simulink model "commhdlQPSKTxRxLoopback"  (R2025b)
settings: Solver=FixedStepDiscrete  StartTime=0.0  StopTime=0.03  RelTol=1e-3
PostLoadFcn:
  | hScopeConfig = get_param([gcs '/Receiver/QPSK Rx/Frequency and Time Synchronizer/Symbol Synchronizer/No HDL/QPSK Receiver Eye Diagram'],'ScopeConfiguration');
  | 
  | hScopeConfig.OpenAtSimulationStart = false;
  | hScopeConfig.Visible = false;
  | SamplesPerSymbol = 4;
  | %UpsamplesRx = 1;
  | clear hScopeConfig
InitFcn:
  | % RxAlign decoder latency (flat_simfix): 41 = netlist value used for HDL; set
  | % rxAlignLat = 25 in the base workspace before a model-level simulation.
  | if ~exist('rxAlignLat','var'), rxAlignLat = uint16(41); end
  | commhdlQPSKTxRxModelInit;
  | % Rate bridge: ADRV9002/Jupiter radio runs at 15.36 MHz = 2x the 7.68 MHz
  | % (4 samples/symbol @ Rsym=1.92 MHz) the QPSK Rx requires. The deployed
  | % Receiver must downsample the ADC stream by 2. UpsamplesRx=1 fed the QPSK
  | % Rx 8 sps (2x-upsampled) and broke symbol sync / the loopback bit check.
  | UpsamplesRx = 1;   %% T8 RATE FIX: rail 15.36e6 == ADC bus rate,
  | %% no ingress decimation (was 2 when the rail sat on the 7.68e6 rung)
  | UpsamplesTx = 1;
  | clear simTimingOffset;
StopFcn:
  | if exist('simTimingOffset','var')
  |   disp('Simulation completed');
  |   %QPSKTxRxVerification;
  | end
undefined symbols (not defined in the file or in its folder): Add, Config, fsym, randsrc, RandStream, Rsym, rxAlignLat, Shift
libraries: hdlsllib x141, simulink x45, dspsigops x30, dsphdlfiltering2 x6, dsphdlsigops2 x4, dsphdlmathfun2 x4, commdigbbndpm3 x4, dspmlti4 x2, commchan3 x1, commrflib2 x1, commcnvcod2 x1
(part 7 of 9)

== system commhdlQPSKTxRxLoopback/TxRxComposite/Receiver/QPSK Rx/Frequency and Time Synchronizer/Symbol Synchronizer/Rate Handle ==
  note: RATE HANDLE -- purpose
      | The Symbol Synchronizer's interpolator emits one symbol per timing-loop strobe, so its output is
      | valid on an IRREGULAR beat (the strobe drifts with the sample-rate offset and the timing correction).
      | Everything downstream (CFC, carrier sync, preamble detector, packet controller, demod) assumes a
      | REGULAR symbol stream: one valid in exactly 4 rail beats (sps = 4).  This block converts the former
      | to the latter with a small FIFO:
      |    push  = strobe            (dataIn is written whenever the interpolator produced a symbol)
      |    pop   = validIn & (phase == 0)   where phase is the free-running mod-4 HDL Counter
      | so validOut/dataOut are a 1-in-4 symbol stream and the FIFO absorbs the jitter between the two rates.
      | If the input runs slow the FIFO drains (EMPTY edge); if it runs fast it fills (FULL edge).  Those two
      | edges are the receiver's only rate-mismatch failure points, which is why every fix and instrument
      | in this subsystem watches or steers the pop.
      | Stock blocks: dataIn, strobe, validIn, Constant, FIFO, HDL Counter, Compare To Constant,
      | Logical Operator, dataOut, validOut.  Everything else was added by the overlay stack (notes below).
  note: bfGridEn / BfGridPace  (beatfix_overlay.m, fixctl 0x208 bit 2)
      | Selects which mod-4 phase counter drives the pop grid.  en = 0: the stock HDL Counter
      | (counts validIn beats).  en = 1: an absolute pacer that counts EVERY rail beat, so the pop
      | grid cannot slip when validIn drops out.  Default off = legacy-identical.
  note: Witness taps (read-only, no effect on the data path)
      | beatobsRhCtr / beatobsPush / beatobsPop  (beatobs_overlay.m): the mod-4 phase pointer and the FIFO
      |    push/pop pointers, routed up to the debug capture bus.
      | w1Strobe / w1Occ / w1PopEmpty / w1PushFull / w1PushPtr / w1PopPtr  (rxfix_w1_overlay.m): the W1 census
      |    inputs.  w1Occ is the FIFO's registered TRUE occupancy (not a pointer delta), counted by RxW1Census
      |    in the Frequency and Time Synchronizer into AXI 0x214-0x230 (0x220 = this block's validOut count).
  note: RxSteer -- pop steering  (rxfix_steer_overlay.m; formerly netlist variants R4B / R4D)
      | Keeps the FIFO away from its EMPTY and FULL edges by editing the pop, once per 13-slot window:
      |    window opens on sroPcEnd (Packet Controller endOut), lock after 8 windows
      |    occ <= 8   -> arm skipEn  : suppress one nominal pop        (EMPTY-edge guard, always on)
      |    occ >= 24  -> arm extraEn : insert one extra pop at phase 2 (FULL-edge guard, only if sroSign = 1)
      |    pop = (popNom & ~skipEn) | (extraEn & validIn & phase2 & sroSign)
      | sroSign is fixctl bit 5: 0 = R4B behaviour (148, negative SRO), 1 = R4D (146, positive SRO).
      | The pop expression is built from the AND/NOT/OR primitives OUTSIDE the MATLAB Function block, and
      | sroPcEnd / occ enter through Delay blocks, so HDL Coder cannot add a delay-match register that
      | would move the pop by a beat.  Witnesses: r4_wit 0x234 {locked, skips, opens}, r4_extras 0x238,
      | sro_mode 0x25C {extraArmed, sroSign}.
  dataIn : Inport
  strobe : Inport  Port=2
  validIn : Inport  Port=3
  bfGridEn : Inport  Port=4  OutDataTypeStr=boolean
  sroPcEnd : Inport  Port=5  OutDataTypeStr=boolean
  sroSign : Inport  Port=6  OutDataTypeStr=boolean
  BfGridPace : MATLAB Function  TreatAsAtomicUnit=on
  Compare To Constant : simulink/Logic and Bit Operations/Compare To Constant  relop===  const=0  OutDataTypeStr=boolean
  Constant : Constant  Value=false  SampleTime=-1
  FIFO : Subsystem  mask{fifoSize=32, pushFullDiag=Error, popEmptyDiag=Ignore}
      mask prompts: fifoSize "FIFO size:"; pushFullDiag "Push full FIFO:"; popEmptyDiag "Pop empty FIFO:"
      mask TypeOptions pushFullDiag: Ignore | Warning | Error
      mask TypeOptions popEmptyDiag: Ignore | Warning | Error
  HDL Counter : hdlsllib/Sources/HDL Counter  CountType=Count limited  CountInit=0  CountStep=1  CountMax=SamplesPerSymbol - 1  CountFromType=Initial value  CountFrom=0  CountResetPort=off  CountLoadPort=off  CountEnbPort=on  CountDirPort=off  CountHitOutputPort=off  CountDataType=Unsigned  CountWordLen=max(1, nextpow2(SamplesPerSymbol - 1))  CountFracLen=0  CountSampTime=1
  Logical Operator : Logic  AllPortsSameDT=off  OutDataTypeStr=boolean
  RxSteer : MATLAB Function  TreatAsAtomicUnit=on
  RxSteerDtcOcc : DataTypeConversion  OutDataTypeStr=uint8  ConvertRealWorld=Stored Integer (SI)  SaturateOnIntegerOverflow=off  RndMeth=Floor
  RxSteerExtraAnd : Logic  Inputs=4  AllPortsSameDT=off  OutDataTypeStr=boolean
  RxSteerNotSkip : Logic  Operator=NOT  Inputs=1  AllPortsSameDT=off  OutDataTypeStr=boolean
  RxSteerOccDly : Delay  DelayLength=1
  RxSteerOccFloor : simulink/Logic and Bit Operations/Compare To Constant  relop=>=  const=2  OutDataTypeStr=boolean
  RxSteerPhase2 : simulink/Logic and Bit Operations/Compare To Constant  relop===  const=1  OutDataTypeStr=boolean
  RxSteerPopOr : Logic  Operator=OR  AllPortsSameDT=off  OutDataTypeStr=boolean
  RxSteerSkipAnd : Logic  Inputs=3  AllPortsSameDT=off  OutDataTypeStr=boolean
  Terminator : Terminator
  dataOut : Outport
  validOut : Outport  Port=2
  beatobsRhCtr : Outport  Port=3
  beatobsPush : Outport  Port=4
  beatobsPop : Outport  Port=5
  w1Strobe : Outport  Port=6
  w1Occ : Outport  Port=7
  w1PopEmpty : Outport  Port=8
  w1PushFull : Outport  Port=9
  w1PushPtr : Outport  Port=10
  w1PopPtr : Outport  Port=11
  r4_wit : Outport  Port=12
  r4_extras : Outport  Port=13
  sro_mode : Outport  Port=14
  wires:
  RxSteerExtraAnd/1 -> RxSteerPopOr/2
  RxSteerNotSkip/1 -> RxSteerSkipAnd/2
  RxSteerOccFloor/1 -> RxSteerSkipAnd/3
  RxSteer/5(sroMode) -> sro_mode/1
  RxSteer/4(r4Extras) -> r4_extras/1
  RxSteerPhase2/1 -> RxSteer/4(phase2), RxSteerExtraAnd/3
  RxSteer/2(extraEn) -> RxSteerExtraAnd/1
  dataIn/1 -> FIFO/1(in)
  RxSteerSkipAnd/1 -> RxSteerPopOr/1
  RxSteerOccDly/1 -> RxSteerDtcOcc/1
  Logical Operator/1 -> RxSteerSkipAnd/1, RxSteer/2(popNom)
  validIn/1 -> HDL Counter/1, RxSteerExtraAnd/2, RxSteer/1(validIn), Logical Operator/1
  BfGridPace/1(y) -> beatobsRhCtr/1, Compare To Constant/1, RxSteerPhase2/1
  FIFO/3(validPop) -> validOut/1
  bfGridEn/1 -> BfGridPace/2(en)
  FIFO/2(numEntries) -> Terminator/1
  FIFO/1(out) -> dataOut/1
  RxSteerPopOr/1 -> FIFO/3(pop)
  Constant/1 -> FIFO/4(reset)
  FIFO/6(w1Occ) -> RxSteerOccDly/1, w1Occ/1
  RxSteer/3(r4Wit) -> r4_wit/1
  HDL Counter/1 -> BfGridPace/1(c)
  FIFO/4(beatobsPush) -> beatobsPush/1
  strobe/1 -> w1Strobe/1, FIFO/2(push)
  FIFO/7(w1PopEmpty) -> w1PopEmpty/1
  FIFO/5(beatobsPop) -> beatobsPop/1
  FIFO/8(w1PushFull) -> w1PushFull/1
  FIFO/9(w1PushPtr) -> w1PushPtr/1
  FIFO/10(w1PopPtr) -> w1PopPtr/1
  sroPcEnd/1 -> RxSteer/5(pcEnd)
  sroSign/1 -> RxSteer/6(sroSign), RxSteerExtraAnd/4
  RxSteerDtcOcc/1 -> RxSteerOccFloor/1, RxSteer/3(occ)
  Compare To Constant/1 -> Logical Operator/2
  RxSteer/1(skipEn) -> RxSteerNotSkip/1

== system commhdlQPSKTxRxLoopback/TxRxComposite/Transmitter/QPSK Tx/Bit Packetizer/Data Bits FIFO/No HDL ==
  push : Inport
  pop : Inport  Port=2
  MATLAB Function : MATLAB Function  TreatAsAtomicUnit=on
  No HDL : Subsystem
  wires:
  MATLAB Function/3(empty) -> No HDL/4(empty)
  MATLAB Function/2(ncount) -> No HDL/3(ncount)
  MATLAB Function/1(full) -> No HDL/2(full)
  pop/1 -> MATLAB Function/2(rd), No HDL/5(pop)
  push/1 -> MATLAB Function/1(wr), No HDL/1(push)

== system commhdlQPSKTxRxLoopback/TxRxComposite/Transmitter/QPSK Tx/Bit Packetizer/Preamble Bits Generator/Preamble Bits Store ==
  note: The Preamble is padded with zeros in the LUT such that
      | the length is the 2^nextpow2(length(Preamble)) for
      | efficient resource mapping to RAM
  actualPreamble : Inport
  sampleCount : Inport  Port=2
  Constant : Constant  OutDataTypeStr=boolean  SampleTime=1/(Rsym*SamplesPerSymbol)
  Extract Bits : simulink/Logic and Bit Operations/Extract Bits  bitsToExtract=Range of bits  numBits=8  bitIdxRange=[0 nextpow2(length(Preamble))-1]  outScalingMode=Treat bit field as an integer
  Preamble : LookupNDDirect  NumberOfTableDimensions=1  Table=[Preamble;false(32-length(Preamble),1)]  DiagnosticForOutOfRangeInput=Error
  Switch : Switch  Criteria=u2 ~= 0  Threshold=1  SaturateOnIntegerOverflow=off  InputSameDT=off
  preamble : Outport
  wires:
  Switch/1 -> preamble/1
  Constant/1 -> Switch/3
  actualPreamble/1 -> Switch/2
  Preamble/1 -> Switch/1
  Extract Bits/1 -> Preamble/1
  sampleCount/1 -> Extract Bits/1

== system commhdlQPSKTxRxLoopback/Receiver/QPSK Rx/Frequency and Time Synchronizer/Coarse Frequency Compensator/Coarse Frequency Estimator/Integrator/Reset Generator ==
  validIn : Inport
  Compare To Constant : simulink/Logic and Bit Operations/Compare To Constant  relop===  const=integAvgLen  OutDataTypeStr=boolean
  Delay1 : Delay  DelayLength=1
  Delay5 : Delay  DelayLength=1
  HDL Counter : hdlsllib/Sources/HDL Counter  CountType=Count limited  CountInit=0  CountStep=1  CountMax=integAvgLen  CountFromType=Initial value  CountFrom=0  CountResetPort=off  CountLoadPort=off  CountEnbPort=on  CountDirPort=off  CountHitOutputPort=off  CountDataType=Unsigned  CountWordLen=nextpow2(integAvgLen + 1)  CountFracLen=0  CountSampTime=1
  Logical Operator : Logic  AllPortsSameDT=off  OutDataTypeStr=boolean
  reset : Outport
  wires:
  Delay1/1 -> Logical Operator/1
  Delay5/1 -> Compare To Constant/1
  Logical Operator/1 -> reset/1
  validIn/1 -> HDL Counter/1, Delay1/1
  Compare To Constant/1 -> Logical Operator/2
  HDL Counter/1 -> Delay5/1

== system commhdlQPSKTxRxLoopback/Receiver/QPSK Rx/Frequency and Time Synchronizer/Phase Ambiguity Estimation and Correction/Phase Ambiguity Corrector/Reciprocal/Function Impl ==
  switch : Inport
  LUTAddr : Inport  Port=2
  Delay{6..8,10,15..16} (6 alike) : Delay
  Delay9 : Delay  DelayLength=1
  LUT1 : LookupNDDirect  NumberOfTableDimensions=1  Table=LUT(:,1)  DiagnosticForOutOfRangeInput=Error
  LUT2 : LookupNDDirect  NumberOfTableDimensions=1  Table=LUT(:,2)  DiagnosticForOutOfRangeInput=Error
  Multiport Switch : MultiPortSwitch  DataPortOrder=Zero-based contiguous  Inputs=2  zeroidx=on  SaturateOnIntegerOverflow=off  InputSameDT=off
  functionValues : Outport
  wires:
  Multiport Switch/1 -> Delay9/1
  Delay6/1 -> LUT1/1
  Delay7/1 -> LUT2/1
  Delay8/1 -> Delay10/1
  switch/1 -> Delay8/1
  LUT1/1 -> Delay16/1
  LUT2/1 -> Delay15/1
  Delay9/1 -> functionValues/1
  Delay10/1 -> Multiport Switch/1
  Delay16/1 -> Multiport Switch/3
  Delay15/1 -> Multiport Switch/2
  LUTAddr/1 -> Delay6/1, Delay7/1

== system commhdlQPSKTxRxLoopback/Receiver/QPSK Rx/Frequency and Time Synchronizer/Preamble Detector/FIFO/Validate Input Push Pop/No HDL ==
  pushFullFIFO : Inport
  popEmptyFIFO : Inport  Port=2
  Constant2 : Constant  Value=pushFullDiag  SampleTime=-1
  Constant3 : Constant  Value=popEmptyDiag  SampleTime=-1
  MATLAB Function : MATLAB Function  TreatAsAtomicUnit=on
  wires:
  Constant2/1 -> MATLAB Function/1(pushFullDiag)
  Constant3/1 -> MATLAB Function/2(popEmptyDiag)
  popEmptyFIFO/1 -> MATLAB Function/4(popEmpty)
  pushFullFIFO/1 -> MATLAB Function/3(pushFull)

== system commhdlQPSKTxRxLoopback/Receiver/QPSK Rx/Frequency and Time Synchronizer/Preamble Detector/Timing Adjust/No HDL/No HDL ==
  timingOffset : Inport
  Enable : EnablePort
  Data Type Conversion : DataTypeConversion  OutDataTypeStr=double  SaturateOnIntegerOverflow=off  RndMeth=Floor
  To Workspace : ToWorkspace  VariableName=simTimingOffset  SampleTime=-1
      settings: Save2DSignal=2-D array (concatenate along first dimension)
  wires:
  Data Type Conversion/1 -> To Workspace/1
  timingOffset/1 -> Data Type Conversion/1

== system commhdlQPSKTxRxLoopback/Receiver/QPSK Rx/Frequency and Time Synchronizer/Preamble Detector/Timing Adjust/No HDL/No HDL1 ==
  frameNumber : Inport
  Enable : EnablePort
  Data Type Conversion : DataTypeConversion  OutDataTypeStr=double  SaturateOnIntegerOverflow=off  RndMeth=Floor
  To Workspace : ToWorkspace  VariableName=simSyncedPackets  SampleTime=-1
      settings: Save2DSignal=2-D array (concatenate along first dimension)
  wires:
  frameNumber/1 -> Data Type Conversion/1
  Data Type Conversion/1 -> To Workspace/1

== system commhdlQPSKTxRxLoopback/Receiver/QPSK Rx/Frequency and Time Synchronizer/Symbol Synchronizer/Rate Handle/FIFO/Validate Input Push Pop ==
  rst : Inport
  push : Inport  Port=2
  pop : Inport  Port=3
  Compare To Constant : hdlsllib/Logic and Bit Operations/Compare To Constant  relop===  const=0  OutDataTypeStr=boolean
  Compare To Constant1 : hdlsllib/Logic and Bit Operations/Compare To Constant  relop===  const=fifoSize  OutDataTypeStr=boolean
  Constant : Constant  Value=true  SampleTime=-1
  Constant1 : Constant  Value=false  SampleTime=-1
  Delay : Delay  DelayLength=1
  Logical Operator1 : Logic  Operator=XOR  AllPortsSameDT=off  OutDataTypeStr=boolean
  Logical Operator2 : Logic  Operator=NOT  AllPortsSameDT=off  OutDataTypeStr=boolean
  Logical Operator{3..5,7,9} (5 alike) : Logic  AllPortsSameDT=off  OutDataTypeStr=boolean
  Logical Operator6 : Logic  Operator=NOT  AllPortsSameDT=off  OutDataTypeStr=boolean
  Logical Operator8 : Logic  Operator=NOT  AllPortsSameDT=off  OutDataTypeStr=boolean
  MATLAB Function : MATLAB Function  TreatAsAtomicUnit=on  mask{initVal=0, countToVal=fifoSize}
      mask prompts: initVal "Initial value:"; countToVal "Count to value:"
  No HDL : Subsystem
  Switch : Switch  Criteria=u2 ~= 0  SaturateOnIntegerOverflow=off  InputSameDT=off
  valid push : Outport
  valid pop : Outport  Port=2
  numEntries : Outport  Port=3
  wires:
  Logical Operator9/1 -> Logical Operator1/1, valid push/1
  Logical Operator2/1 -> Logical Operator9/2
  Logical Operator5/1 -> Logical Operator4/1
  Logical Operator8/1 -> Logical Operator5/2
  push/1 -> Logical Operator5/1, Logical Operator9/1
  Logical Operator1/1 -> MATLAB Function/2(enb)
  Logical Operator6/1 -> Logical Operator7/2
  Logical Operator7/1 -> Switch/2, valid pop/1, Logical Operator8/1, Logical Operator1/2
  Compare To Constant1/1 -> Logical Operator4/2
  Constant/1 -> Switch/3
  Logical Operator4/1 -> No HDL/1(pushFullFIFO), Logical Operator2/1  "push on full FIFO"
  Logical Operator3/1 -> No HDL/2(popEmptyFIFO), Logical Operator6/1  "pop on empty FIFO"
  Constant1/1 -> Switch/1
  MATLAB Function/1(count) -> Delay/1
  Switch/1 -> MATLAB Function/3(dir)
  pop/1 -> Logical Operator3/2, Logical Operator7/1
  Compare To Constant/1 -> Logical Operator3/1
  rst/1 -> MATLAB Function/1(rst)
  Delay/1 -> Compare To Constant1/1, numEntries/1, Compare To Constant/1

== system commhdlQPSKTxRxLoopback/TxRxComposite/Receiver/QPSK Rx/Frequency and Time Synchronizer/Coarse Frequency Compensator/Coarse Frequency Estimator/Extract Frequency ==
  datain : Inport
  validIn : Inport  Port=2
  Complex to Magnitude-Angle HDL Optimized : dsphdlmathfun2/Complex to Magnitude-Angle  NumIterationsSource=Auto  NumIterations=10  OutputFormat=Angle  AngleFormat=Normalized  ScaleOutput=on  ScalingMethod=Shift-Add  SimulateUsing=Code generation
  Delay{1..4} (4 alike) : Delay  DelayLength=1
  Gain : Gain  Gain=1/2  ParamDataTypeStr=fixdt(0,1,1)  OutDataTypeStr=Inherit: Same as input
  Unit Delay Enabled Synchronous : hdlsllib/Discrete/Unit Delay Enabled Synchronous  InitialCondition=0.0  SampleTime=-1
  normFreqOut : Outport
  wires:
  Delay3/1 -> normFreqOut/1
  Gain/1 -> Delay3/1
  Delay2/1 -> Gain/1
  Unit Delay Enabled Synchronous/1 -> Delay2/1
  Complex to Magnitude-Angle HDL Optimized/2 -> Unit Delay Enabled Synchronous/2
  Complex to Magnitude-Angle HDL Optimized/1 -> Unit Delay Enabled Synchronous/1
  Delay4/1 -> Complex to Magnitude-Angle HDL Optimized/2
  validIn/1 -> Delay4/1
  Delay1/1 -> Complex to Magnitude-Angle HDL Optimized/1
  datain/1 -> Delay1/1

== system commhdlQPSKTxRxLoopback/TxRxComposite/Receiver/QPSK Rx/Frequency and Time Synchronizer/Coarse Frequency Compensator/Coarse Frequency Estimator/Integrator ==
  note: store the value in the Reg before reset
  dataIn : Inport
  validIn : Inport  Port=2
  Add1 : Sum  Inputs=|++  OutDataTypeStr=Inherit: Same as first input
  Delay : Delay  DelayLength=1
  Delay1 : Delay  DelayLength=1
  Delay2 : Delay  DelayLength=1
  Integ Reg : hdlsllib/Discrete/Unit Delay Enabled Resettable Synchronous  InitialCondition=0.0  SampleTime=-1
  Reset Generator : Subsystem
  Store Reg : hdlsllib/Discrete/Unit Delay Enabled Synchronous  InitialCondition=0.0  SampleTime=-1
  IntegOut : Outport
  IntegValid : Outport  Port=2
  wires:
  Add1/1 -> Integ Reg/1
  Store Reg/1 -> IntegOut/1
  Delay1/1 -> Add1/1
  Delay/1 -> IntegValid/1
  Integ Reg/1 -> Store Reg/1, Add1/2
  Delay2/1 -> Integ Reg/2
  dataIn/1 -> Delay1/1
  Reset Generator/1(reset) -> Integ Reg/3, Delay/1, Store Reg/2
  validIn/1 -> Delay2/1, Reset Generator/1(validIn)

== system commhdlQPSKTxRxLoopback/TxRxComposite/Receiver/QPSK Rx/Frequency and Time Synchronizer/Phase Ambiguity Estimation and Correction/Phase Ambiguity Corrector/Reciprocal ==
  dataIn : Inport
  Compare To Constant : simulink/Logic and Bit Operations/Compare To Constant  relop=<  const=0  OutDataTypeStr=boolean
  Data Type Conversion : DataTypeConversion  OutDataTypeStr=fixdt(1,WL,0)  ConvertRealWorld=Stored Integer (SI)  SaturateOnIntegerOverflow=off  RndMeth=Floor
  Data Type Conversion1 : DataTypeConversion  OutDataTypeStr=fixdt(0,LUTAddrWL,0)  ConvertRealWorld=Stored Integer (SI)  SaturateOnIntegerOverflow=off  RndMeth=Floor
  Data Type Conversion2 : DataTypeConversion  OutDataTypeStr=fixdt(0,WL-LUTAddrWL,0)  ConvertRealWorld=Stored Integer (SI)  SaturateOnIntegerOverflow=off  RndMeth=Floor
  Delay : Delay  DelayLength=1
  Delay1 : Delay  DelayLength=1
  Delay2 : Delay  DelayLength=1
  Extract Bits : simulink/Logic and Bit Operations/Extract Bits  bitsToExtract=Range ending with least significant bit  numBits=LUTAddrWL  bitIdxRange=[0 7]  outScalingMode=Treat bit field as an integer
  Function Impl : Subsystem
  dataOut : Outport
  wires:
  Data Type Conversion1/1 -> Function Impl/2(LUTAddr)
  Data Type Conversion2/1 -> Function Impl/1(switch)
  Delay2/1 -> Data Type Conversion1/1
  Delay1/1 -> Data Type Conversion2/1
  Function Impl/1(functionValues) -> dataOut/1
  Delay/1 -> Compare To Constant/1, Extract Bits/1
  Compare To Constant/1 -> Delay1/1
  Data Type Conversion/1 -> Delay/1
  Extract Bits/1 -> Delay2/1
  dataIn/1 -> Data Type Conversion/1

== system commhdlQPSKTxRxLoopback/TxRxComposite/Receiver/QPSK Rx/Frequency and Time Synchronizer/Phase Ambiguity Estimation and Correction/Phase Ambiguity Estimator/Subsystem ==
  L : Inport
  H : Inport  Port=2
  Delay6 : Delay  DelayLength=1  InitialCondition=1
  Logical Operator : Logic  AllPortsSameDT=off  OutDataTypeStr=boolean
  Logical Operator1 : Logic  Operator=NOT  IconShape=distinctive  AllPortsSameDT=off  OutDataTypeStr=boolean
  Logical Operator2 : Logic  Operator=OR  AllPortsSameDT=off  OutDataTypeStr=boolean
  Out2 : Outport
  wires:
  Logical Operator/1 -> Logical Operator2/2
  Delay6/1 -> Out2/1, Logical Operator/2
  Logical Operator1/1 -> Logical Operator/1
  Logical Operator2/1 -> Delay6/1
  L/1 -> Logical Operator1/1
  H/1 -> Logical Operator2/1

== system commhdlQPSKTxRxLoopback/TxRxComposite/Receiver/QPSK Rx/Frequency and Time Synchronizer/Phase Ambiguity Estimation and Correction/Phase Ambiguity Estimator/Subsystem1 ==
  In1 : Inport
  validIn : Inport  Port=2
  Logical Operator1 : Logic  IconShape=distinctive  AllPortsSameDT=off  OutDataTypeStr=boolean
  Logical Operator2 : Logic  Operator=NOT  IconShape=distinctive  AllPortsSameDT=off  OutDataTypeStr=boolean
  validOut : Outport
  wires:
  validIn/1 -> Logical Operator1/2
  Logical Operator1/1 -> validOut/1
  Logical Operator2/1 -> Logical Operator1/1
  In1/1 -> Logical Operator2/1

== system commhdlQPSKTxRxLoopback/TxRxComposite/Receiver/QPSK Rx/Frequency and Time Synchronizer/Preamble Detector/Correlator/Magnitude Squared ==
  In1 : Inport
  Delay1 : Delay
  Delay2 : Delay
  Delay3 : Delay
  Math Function : Math  Operator=conj
  Product : Product
  Out1 : Outport
  wires:
  Delay3/1 -> Out1/1
  Product/1 -> Delay3/1
  Delay1/1 -> Product/2
  Delay2/1 -> Product/1
  Math Function/1 -> Delay1/1
  In1/1 -> Math Function/1, Delay2/1

== system commhdlQPSKTxRxLoopback/TxRxComposite/Receiver/QPSK Rx/Frequency and Time Synchronizer/Preamble Detector/Correlator/Magnitude Squared and Moving Sum ==
  scaled1 : Inport
  validIn : Inport  Port=2
  Add : Sum  Inputs=|+-  OutDataTypeStr=Inherit: Same as first input
  Add1 : Sum  Inputs=|++  OutDataTypeStr=Inherit: Same as first input
  Complex to Real-Imag1 : ComplexToRealImag  Output=Real
  Delay : Delay  DelayLength=26  ShowEnablePort=on
      settings: InputPortMap=u0,e6
  Delay{1..4,6,8..10,12} (9 alike) : Delay
  Delay11 : Delay  DelayLength=24
  Delay14 : Delay  DelayLength=1  ShowEnablePort=on
      settings: InputPortMap=u0,e6
  Delay5 : Delay  DelayLength=1
  Delay7 : Delay  DelayLength=1
  Gain : Gain  Gain=ThresoldGainFac  OutDataTypeStr=Inherit: Same as input
  Math Function1 : Math  Operator=conj
  Product1 : Product
  E1 : Outport
  wires:
  Delay11/1 -> E1/1
  Delay5/1 -> Add1/1
  Add/1 -> Delay5/1
  Delay/1 -> Add/2
  Delay4/1 -> Delay/1, Add/1
  Delay8/1 -> Delay/2, Delay7/1
  scaled1/1 -> Math Function1/1, Delay6/1
  Gain/1 -> Delay4/1
  validIn/1 -> Delay12/1
  Delay6/1 -> Product1/1
  Delay7/1 -> Delay14/2
  Math Function1/1 -> Delay1/1
  Product1/1 -> Delay2/1
  Delay10/1 -> Delay9/1
  Delay3/1 -> Gain/1
  Add1/1 -> Delay11/1, Delay14/1
  Delay1/1 -> Product1/2
  Delay14/1 -> Add1/2
  Delay9/1 -> Delay8/1
  Delay2/1 -> Complex to Real-Imag1/1
  Complex to Real-Imag1/1 -> Delay3/1
  Delay12/1 -> Delay10/1

== system commhdlQPSKTxRxLoopback/TxRxComposite/Receiver/QPSK Rx/Frequency and Time Synchronizer/Preamble Detector/FIFO/Validate Input Push Pop ==
  rst : Inport
  push : Inport  Port=2
  pop : Inport  Port=3
  Compare To Constant : hdlsllib/Logic and Bit Operations/Compare To Constant  relop===  const=0  OutDataTypeStr=boolean
  Compare To Constant1 : hdlsllib/Logic and Bit Operations/Compare To Constant  relop===  const=fifoSize  OutDataTypeStr=boolean
  Constant : Constant  Value=true  SampleTime=-1
  Constant1 : Constant  Value=false  SampleTime=-1
  Delay : Delay  DelayLength=1
  Logical Operator1 : Logic  Operator=XOR  AllPortsSameDT=off  OutDataTypeStr=boolean
  Logical Operator2 : Logic  Operator=NOT  AllPortsSameDT=off  OutDataTypeStr=boolean
  Logical Operator{3..5,7,9} (5 alike) : Logic  AllPortsSameDT=off  OutDataTypeStr=boolean
  Logical Operator6 : Logic  Operator=NOT  AllPortsSameDT=off  OutDataTypeStr=boolean
  Logical Operator8 : Logic  Operator=NOT  AllPortsSameDT=off  OutDataTypeStr=boolean
  MATLAB Function : MATLAB Function  TreatAsAtomicUnit=on  mask{initVal=0, countToVal=fifoSize}
      mask prompts: initVal "Initial value:"; countToVal "Count to value:"
  No HDL : Subsystem
  Switch : Switch  Criteria=u2 ~= 0  SaturateOnIntegerOverflow=off  InputSameDT=off
  valid push : Outport
  valid pop : Outport  Port=2
  numEntries : Outport  Port=3
  wires:
  Logical Operator3/1 -> No HDL/2(popEmptyFIFO), Logical Operator6/1  "pop on empty FIFO"
  Logical Operator4/1 -> No HDL/1(pushFullFIFO), Logical Operator2/1  "push on full FIFO"
  Compare To Constant/1 -> Logical Operator3/1
  Compare To Constant1/1 -> Logical Operator4/2
  Delay/1 -> Compare To Constant/1, Compare To Constant1/1, numEntries/1
  Logical Operator6/1 -> Logical Operator7/2
  push/1 -> Logical Operator9/1, Logical Operator5/1
  Logical Operator1/1 -> MATLAB Function/2(enb)
  Constant1/1 -> Switch/1
  pop/1 -> Logical Operator7/1, Logical Operator3/2
  rst/1 -> MATLAB Function/1(rst)
  Logical Operator8/1 -> Logical Operator5/2
  Switch/1 -> MATLAB Function/3(dir)
  Logical Operator2/1 -> Logical Operator9/2
  Logical Operator7/1 -> Switch/2, Logical Operator8/1, valid pop/1, Logical Operator1/2
  Logical Operator9/1 -> Logical Operator1/1, valid push/1
  MATLAB Function/1(count) -> Delay/1
  Constant/1 -> Switch/3
  Logical Operator5/1 -> Logical Operator4/1

== system commhdlQPSKTxRxLoopback/TxRxComposite/Receiver/QPSK Rx/Frequency and Time Synchronizer/Preamble Detector/Timing Adjust/No HDL ==
  note: This subsystem generates variables required for QPSKRxVerification for validation
  validIn : Inport
  timingOffset : Inport  Port=2
  syncPulse : Inport  Port=3
  Compare To Constant : simulink/Logic and Bit Operations/Compare To Constant  relop===  const=0  OutDataTypeStr=boolean
  Delay : Delay  DelayLength=4
  Delay1 : Delay  DelayLength=4
  Frame Counter : hdlsllib/Sources/HDL Counter  CountType=Free running  CountInit=0  CountStep=1  CountMax=bitsPerPacket/2 - 1  CountFromType=Initial value  CountFrom=0  CountResetPort=off  CountLoadPort=off  CountEnbPort=on  CountDirPort=off  CountHitOutputPort=off  CountDataType=Unsigned  CountWordLen=32  CountFracLen=0  CountSampTime=1
  Logical Operator : Logic  AllPortsSameDT=off  OutDataTypeStr=boolean
  No HDL : Subsystem
  No HDL1 : Subsystem
  Symbol Counter : hdlsllib/Sources/HDL Counter  CountType=Count limited  CountInit=0  CountStep=1  CountMax=bitsPerPacket/2 - 1  CountFromType=Initial value  CountFrom=0  CountResetPort=off  CountLoadPort=off  CountEnbPort=on  CountDirPort=off  CountHitOutputPort=off  CountDataType=Unsigned  CountWordLen=nextpow2(bitsPerPacket/2 - 1)  CountFracLen=0  CountSampTime=1
  Unit Delay Enabled Synchronous : hdlsllib/Discrete/Unit Delay Enabled Synchronous  InitialCondition=0.0  SampleTime=-1
  wires:
  Delay/1 -> No HDL1/Enable, No HDL/Enable
  Delay1/1 -> No HDL/1(timingOffset)
  timingOffset/1 -> Delay1/1
  Unit Delay Enabled Synchronous/1 -> No HDL1/1(frameNumber)
  Frame Counter/1 -> Unit Delay Enabled Synchronous/1
  Logical Operator/1 -> Frame Counter/1, Unit Delay Enabled Synchronous/2
  Symbol Counter/1 -> Compare To Constant/1
  syncPulse/1 -> Delay/1
  Compare To Constant/1 -> Logical Operator/1
  validIn/1 -> Symbol Counter/1, Logical Operator/2

== system commhdlQPSKTxRxLoopback/TxRxComposite/Receiver/QPSK Rx/Frequency and Time Synchronizer/Symbol Synchronizer/Gardner TED/GTED ==
  In1 : Inport
  Add : Sum
  Add1 : Sum  Inputs=+-
  Add2 : Sum  Inputs=+-
  Complex to Real-Imag : ComplexToRealImag
  Delay{,1,4..5,8,11} (6 alike) : Delay  DelayLength=1
  Delay{9..10,12..13} (4 alike) : Delay
  Product : Product
  Product1 : Product
  Out1 : Outport
  wires:
  Add/1 -> Out1/1
  Delay13/1 -> Add/2
  Delay10/1 -> Add/1
  Product/1 -> Delay10/1
  Complex to Real-Imag/2 -> Delay4/1, Add2/2
  Delay8/1 -> Product/1
  Add1/1 -> Delay9/1
  Delay/1 -> Delay1/1
  Product1/1 -> Delay13/1
  In1/1 -> Complex to Real-Imag/1
  Delay4/1 -> Delay5/1
  Delay1/1 -> Delay8/1, Add1/1
  Delay5/1 -> Add2/1, Delay11/1
  Add2/1 -> Delay12/1
  Delay9/1 -> Product/2
  Delay11/1 -> Product1/1
  Complex to Real-Imag/1 -> Delay/1, Add1/2
  Delay12/1 -> Product1/2

== system commhdlQPSKTxRxLoopback/TxRxComposite/Receiver/QPSK Rx/Frequency and Time Synchronizer/Symbol Synchronizer/No HDL/No HDL ==
  data : Inport
  Enable : EnablePort
  Data Type Conversion : DataTypeConversion  OutDataTypeStr=double  SaturateOnIntegerOverflow=off  RndMeth=Floor
  wires:
  Data Type Conversion/1 -> ?
  data/1 -> Data Type Conversion/1

== system commhdlQPSKTxRxLoopback/TxRxComposite/Receiver/QPSK Rx/Frequency and Time Synchronizer/Symbol Synchronizer/Rate Handle/FIFO ==
  in : Inport
  push : Inport  Port=2
  pop : Inport  Port=3
  reset : Inport  Port=4
  Delay1 : Delay  DelayLength=1
  Pop Counter : hdlsllib/Sources/HDL Counter  CountType=Count limited  CountInit=0  CountStep=1  CountMax=fifoSize -1  CountFromType=Initial value  CountFrom=0  CountResetPort=on  CountLoadPort=off  CountEnbPort=on  CountDirPort=off  CountHitOutputPort=off  CountDataType=Unsigned  CountWordLen=nextpow2(fifoSize)  CountFracLen=0  CountSampTime=1
  Push Counter : hdlsllib/Sources/HDL Counter  CountType=Count limited  CountInit=0  CountStep=1  CountMax=fifoSize -1  CountFromType=Initial value  CountFrom=0  CountResetPort=on  CountLoadPort=off  CountEnbPort=on  CountDirPort=off  CountHitOutputPort=off  CountDataType=Unsigned  CountWordLen=nextpow2(fifoSize)  CountFracLen=0  CountSampTime=1
  Simple Dual Port RAM : hdlsllib/HDL RAMs/Simple Dual Port RAM  ram_size=nextpow2(fifoSize)
  Validate Input Push Pop : Subsystem
  out : Outport
  numEntries : Outport  Port=2
  validPop : Outport  Port=3
  beatobsPush : Outport  Port=4
  beatobsPop : Outport  Port=5
  w1Occ : Outport  Port=6
  w1PopEmpty : Outport  Port=7
  w1PushFull : Outport  Port=8
  w1PushPtr : Outport  Port=9
  w1PopPtr : Outport  Port=10
  wires:
  Simple Dual Port RAM/1 -> out/1
  reset/1 -> Validate Input Push Pop/1(rst), Delay1/1
  Validate Input Push Pop/6(w1PushFull) -> w1PushFull/1
  push/1 -> Validate Input Push Pop/2(push)
  pop/1 -> Validate Input Push Pop/3(pop)
  Delay1/1 -> Push Counter/1, Pop Counter/1
  Validate Input Push Pop/3(numEntries) -> numEntries/1
  Validate Input Push Pop/1(valid push) -> Push Counter/2, Simple Dual Port RAM/3
  Validate Input Push Pop/4(w1Occ) -> w1Occ/1
  Validate Input Push Pop/5(w1PopEmpty) -> w1PopEmpty/1
  Validate Input Push Pop/2(valid pop) -> Pop Counter/2, validPop/1
  Push Counter/1 -> w1PushPtr/1, beatobsPush/1, Simple Dual Port RAM/2
  Pop Counter/1 -> w1PopPtr/1, beatobsPop/1, Simple Dual Port RAM/4
  in/1 -> Simple Dual Port RAM/1

== system commhdlQPSKTxRxLoopback/TxRxComposite/Transmitter/QPSK Tx/Bit Packetizer/Data Bits FIFO/No HDL/No HDL ==
  push : Inport
  full : Inport  Port=2
  ncount : Inport  Port=3
  empty : Inport  Port=4
  pop : Inport  Port=5
  Assertion : Assertion
  Assertion1 : Assertion
  Display : Display
  Logical Operator : Logic  Operator=NAND  AllPortsSameDT=off  OutDataTypeStr=boolean
  Logical Operator1 : Logic  Operator=NAND  AllPortsSameDT=off  OutDataTypeStr=boolean
  wires:
  Logical Operator1/1 -> Assertion1/1
  pop/1 -> Logical Operator1/2
  Logical Operator/1 -> Assertion/1
  empty/1 -> Logical Operator1/1
  full/1 -> Logical Operator/2
  push/1 -> Logical Operator/1
  ncount/1 -> Display/1

== system commhdlQPSKTxRxLoopback/Receiver/QPSK Rx/Frequency and Time Synchronizer/Symbol Synchronizer/Rate Handle/FIFO/Validate Input Push Pop/No HDL ==
  pushFullFIFO : Inport
  popEmptyFIFO : Inport  Port=2
  Constant2 : Constant  Value=pushFullDiag  SampleTime=-1
  Constant3 : Constant  Value=popEmptyDiag  SampleTime=-1
  MATLAB Function : MATLAB Function  TreatAsAtomicUnit=on
  wires:
  Constant2/1 -> MATLAB Function/1(pushFullDiag)
  Constant3/1 -> MATLAB Function/2(popEmptyDiag)
  popEmptyFIFO/1 -> MATLAB Function/4(popEmpty)
  pushFullFIFO/1 -> MATLAB Function/3(pushFull)

== system commhdlQPSKTxRxLoopback/TxRxComposite/Receiver/QPSK Rx/Frequency and Time Synchronizer/Coarse Frequency Compensator/Coarse Frequency Estimator/Integrator/Reset Generator ==
  validIn : Inport
  Compare To Constant : simulink/Logic and Bit Operations/Compare To Constant  relop===  const=integAvgLen  OutDataTypeStr=boolean
  Delay1 : Delay  DelayLength=1
  Delay5 : Delay  DelayLength=1
  HDL Counter : hdlsllib/Sources/HDL Counter  CountType=Count limited  CountInit=0  CountStep=1  CountMax=integAvgLen  CountFromType=Initial value  CountFrom=0  CountResetPort=off  CountLoadPort=off  CountEnbPort=on  CountDirPort=off  CountHitOutputPort=off  CountDataType=Unsigned  CountWordLen=nextpow2(integAvgLen + 1)  CountFracLen=0  CountSampTime=1
  Logical Operator : Logic  AllPortsSameDT=off  OutDataTypeStr=boolean
  reset : Outport
  wires:
  Logical Operator/1 -> reset/1
  Delay5/1 -> Compare To Constant/1
  Compare To Constant/1 -> Logical Operator/2
  Delay1/1 -> Logical Operator/1
  HDL Counter/1 -> Delay5/1
  validIn/1 -> HDL Counter/1, Delay1/1

== system commhdlQPSKTxRxLoopback/TxRxComposite/Receiver/QPSK Rx/Frequency and Time Synchronizer/Phase Ambiguity Estimation and Correction/Phase Ambiguity Corrector/Reciprocal/Function Impl ==
  switch : Inport
  LUTAddr : Inport  Port=2
  Delay{6..8,10,15..16} (6 alike) : Delay
  Delay9 : Delay  DelayLength=1
  LUT1 : LookupNDDirect  NumberOfTableDimensions=1  Table=LUT(:,1)  DiagnosticForOutOfRangeInput=Error
  LUT2 : LookupNDDirect  NumberOfTableDimensions=1  Table=LUT(:,2)  DiagnosticForOutOfRangeInput=Error
  Multiport Switch : MultiPortSwitch  DataPortOrder=Zero-based contiguous  Inputs=2  zeroidx=on  SaturateOnIntegerOverflow=off  InputSameDT=off
  functionValues : Outport
  wires:
  Delay9/1 -> functionValues/1
  Delay10/1 -> Multiport Switch/1
  LUT1/1 -> Delay16/1
  LUT2/1 -> Delay15/1
  Delay8/1 -> Delay10/1
  Multiport Switch/1 -> Delay9/1
  Delay6/1 -> LUT1/1
  Delay16/1 -> Multiport Switch/3
  Delay15/1 -> Multiport Switch/2
  Delay7/1 -> LUT2/1
  switch/1 -> Delay8/1
  LUTAddr/1 -> Delay6/1, Delay7/1

== system commhdlQPSKTxRxLoopback/TxRxComposite/Receiver/QPSK Rx/Frequency and Time Synchronizer/Preamble Detector/FIFO/Validate Input Push Pop/No HDL ==
  pushFullFIFO : Inport
  popEmptyFIFO : Inport  Port=2
  Constant2 : Constant  Value=pushFullDiag  SampleTime=-1
  Constant3 : Constant  Value=popEmptyDiag  SampleTime=-1
  MATLAB Function : MATLAB Function  TreatAsAtomicUnit=on
  wires:
  pushFullFIFO/1 -> MATLAB Function/3(pushFull)
  popEmptyFIFO/1 -> MATLAB Function/4(popEmpty)
  Constant3/1 -> MATLAB Function/2(popEmptyDiag)
  Constant2/1 -> MATLAB Function/1(pushFullDiag)

== system commhdlQPSKTxRxLoopback/TxRxComposite/Receiver/QPSK Rx/Frequency and Time Synchronizer/Preamble Detector/Timing Adjust/No HDL/No HDL ==
  timingOffset : Inport
  Enable : EnablePort
  Data Type Conversion : DataTypeConversion  OutDataTypeStr=double  SaturateOnIntegerOverflow=off  RndMeth=Floor
  wires:
  timingOffset/1 -> Data Type Conversion/1

== system commhdlQPSKTxRxLoopback/TxRxComposite/Receiver/QPSK Rx/Frequency and Time Synchronizer/Preamble Detector/Timing Adjust/No HDL/No HDL1 ==
  frameNumber : Inport
  Enable : EnablePort
  Data Type Conversion : DataTypeConversion  OutDataTypeStr=double  SaturateOnIntegerOverflow=off  RndMeth=Floor
  wires:
  frameNumber/1 -> Data Type Conversion/1

== system commhdlQPSKTxRxLoopback/TxRxComposite/Receiver/QPSK Rx/Frequency and Time Synchronizer/Symbol Synchronizer/Rate Handle/FIFO/Validate Input Push Pop ==
  rst : Inport
  push : Inport  Port=2
  pop : Inport  Port=3
  Compare To Constant : hdlsllib/Logic and Bit Operations/Compare To Constant  relop===  const=0  OutDataTypeStr=boolean
  Compare To Constant1 : hdlsllib/Logic and Bit Operations/Compare To Constant  relop===  const=fifoSize  OutDataTypeStr=boolean
  Constant : Constant  Value=true  SampleTime=-1
  Constant1 : Constant  Value=false  SampleTime=-1
  Delay : Delay  DelayLength=1
  Logical Operator1 : Logic  Operator=XOR  AllPortsSameDT=off  OutDataTypeStr=boolean
  Logical Operator2 : Logic  Operator=NOT  AllPortsSameDT=off  OutDataTypeStr=boolean
  Logical Operator{3..5,7,9} (5 alike) : Logic  AllPortsSameDT=off  OutDataTypeStr=boolean
  Logical Operator6 : Logic  Operator=NOT  AllPortsSameDT=off  OutDataTypeStr=boolean
  Logical Operator8 : Logic  Operator=NOT  AllPortsSameDT=off  OutDataTypeStr=boolean
  MATLAB Function : MATLAB Function  TreatAsAtomicUnit=on  mask{initVal=0, countToVal=fifoSize}
      mask prompts: initVal "Initial value:"; countToVal "Count to value:"
  No HDL : Subsystem
  Switch : Switch  Criteria=u2 ~= 0  SaturateOnIntegerOverflow=off  InputSameDT=off
  valid push : Outport
  valid pop : Outport  Port=2
  numEntries : Outport  Port=3
  w1Occ : Outport  Port=4
  w1PopEmpty : Outport  Port=5
  w1PushFull : Outport  Port=6
  wires:
  Compare To Constant/1 -> Logical Operator3/1
  Logical Operator4/1 -> w1PushFull/1, No HDL/1(pushFullFIFO), Logical Operator2/1  "push on full FIFO"
  Delay/1 -> w1Occ/1, Compare To Constant/1, Compare To Constant1/1, numEntries/1
  Logical Operator6/1 -> Logical Operator7/2
  Logical Operator3/1 -> w1PopEmpty/1, No HDL/2(popEmptyFIFO), Logical Operator6/1  "pop on empty FIFO"
  push/1 -> Logical Operator9/1, Logical Operator5/1
  Logical Operator5/1 -> Logical Operator4/1
  pop/1 -> Logical Operator7/1, Logical Operator3/2
  Logical Operator9/1 -> Logical Operator1/1, valid push/1
  Logical Operator7/1 -> Switch/2, valid pop/1, Logical Operator1/2, Logical Operator8/1
  Constant1/1 -> Switch/1
  Constant/1 -> Switch/3
  rst/1 -> MATLAB Function/1(rst)
  Compare To Constant1/1 -> Logical Operator4/2
  Logical Operator1/1 -> MATLAB Function/2(enb)
  Logical Operator2/1 -> Logical Operator9/2
  Switch/1 -> MATLAB Function/3(dir)
  Logical Operator8/1 -> Logical Operator5/2
  MATLAB Function/1(count) -> Delay/1

== system commhdlQPSKTxRxLoopback/TxRxComposite/Receiver/QPSK Rx/Frequency and Time Synchronizer/Symbol Synchronizer/Rate Handle/FIFO/Validate Input Push Pop/No HDL ==
  pushFullFIFO : Inport
  popEmptyFIFO : Inport  Port=2
  Constant2 : Constant  Value=pushFullDiag  SampleTime=-1
  Constant3 : Constant  Value=popEmptyDiag  SampleTime=-1
  MATLAB Function : MATLAB Function  TreatAsAtomicUnit=on
  wires:
  pushFullFIFO/1 -> MATLAB Function/3(pushFull)
  popEmptyFIFO/1 -> MATLAB Function/4(popEmpty)
  Constant3/1 -> MATLAB Function/2(popEmptyDiag)
  Constant2/1 -> MATLAB Function/1(pushFullDiag)

== matlab function commhdlQPSKTxRxLoopback/Receiver/QPSK Rx/Frequency and Time Synchronizer/Symbol Synchronizer/Rate Handle/FIFO/Validate Input Push Pop/No HDL/MATLAB Function ==
  data: pushFullDiag input; popEmptyDiag input; pushFull input; popEmpty input
function pushPopDiagnostics(pushFullDiag, popEmptyDiag, pushFull, popEmpty)
%#codegen


if(pushFull)
    switch pushFullDiag
        case 2
            warning('Push signal applied on full FIFO');
        case 3
            error('Push signal applied on full FIFO');
        otherwise
    end
end

if(popEmpty)
    switch popEmptyDiag
        case 2
            warning('Pop signal applied on empty FIFO');
        case 3
            error('Pop signal applied on empty FIFO');
        otherwise
    end
end

end

== matlab function commhdlQPSKTxRxLoopback/Receiver/Capture Data Bits/MATLAB Function ==
  data: valid input; datain input; start input; stop input; count_out output; packets_out output; bit_errors_out output
function [count_out, packets_out, bit_errors_out] = msgdec(valid, datain, start, stop)

persistent count;
persistent msgbuffer;

persistent packetsReceived
persistent errors;

if isempty(count) || isempty(msgbuffer) || isempty(packetsReceived)
    count = uint32(0);
    msgbuffer = zeros(1,120+8)>0; % ADI Hello WorldX
    packetsReceived = uint32(0);
    errors = uint32(0);
end

% Mesg
strAscii = dec2bin('ADI Hello World',8);
msgarray = reshape(strAscii', [1, numel(strAscii)]);
msgbits = logical(msgarray - 48);

% msgLen = uint32(2240);

if valid
    if start
        count = uint32(1);
        packetsReceived = packetsReceived + 1;
    end

    if count <= (length(msgbuffer) - 8)
        msgbuffer(count) = datain;
        if datain ~= msgbits(count)
            errors = errors + 1;
        end

    elseif count == length(msgbuffer) + 1
        msgarray_dec = char('0' + msgbuffer);
        N = length(msgarray_dec) / 8;
        strAscii_dec = reshape(msgarray_dec , 8, N).';
        msg = char(bin2dec(strAscii_dec).');
        disp(msg);
    end
    
    if count <= length(msgbuffer) + 2
        count = count + 1;
    end
end

count_out = count;
packets_out = packetsReceived;
bit_errors_out = errors;
